simulink model "HW3"  (R2023b)
settings: Solver=VariableStepAuto  StartTime=0.0  StopTime=100  FixedStep=0.5  RelTol=1e-3
settings Model: Creator=ArshiaGosh  LastModifiedBy=ArshiaGosh

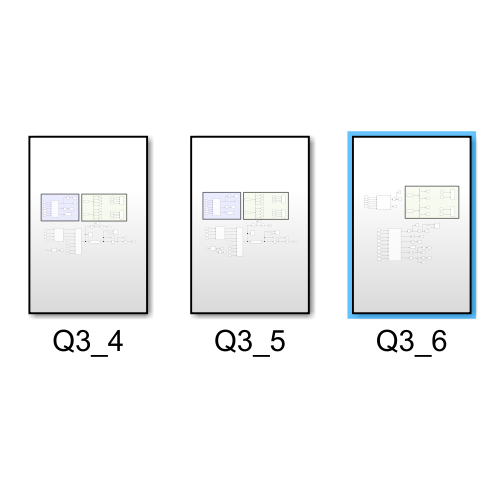
[thumbnail: Simulink's stored preview of the top-level diagram]
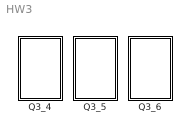
== system HW3 ==
  Q3_4 : Subsystem
  Q3_5 : Subsystem
  Q3_6 : Subsystem

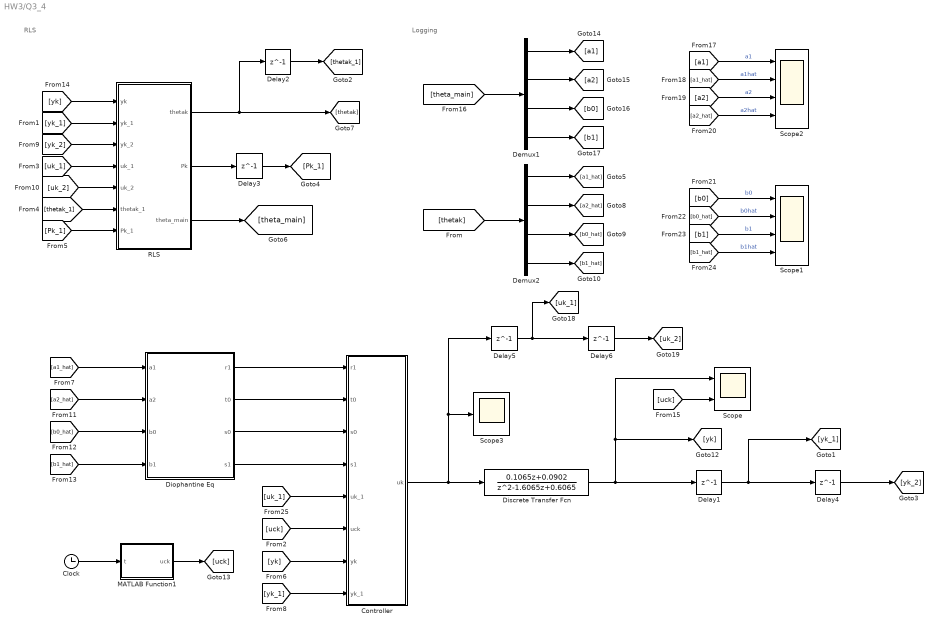
== system HW3/Q3_4 ==
  note: Logging
  note: RLS
  Clock : Clock
  Controller : MATLAB Function  TreatAsAtomicUnit=on
  Delay{1,4..6} (4 alike) : Delay  DelayLength=1
  Delay2 : Delay  DelayLength=1  InitialCondition=[0;0;0.01;0.2]
  Delay3 : Delay  DelayLength=1  InitialCondition=[100 0 0 0;0 100 0 0;0 0 1 0;0 0 0 1]
  Demux1 : Demux
  Demux2 : Demux
  Diophantine Eq : MATLAB Function  TreatAsAtomicUnit=on
  Discrete Transfer Fcn : DiscreteTransferFcn  Numerator=[0.1065 0.0902]  Denominator=[1 -1.6065 0.6065]
  MATLAB Function1 : MATLAB Function  TreatAsAtomicUnit=on
  RLS : MATLAB Function  TreatAsAtomicUnit=on
  Scope : Scope  NumInputPorts=2
  Scope1 : Scope  NumInputPorts=4
  Scope2 : Scope  NumInputPorts=4
  Scope3 : Scope
  wires:
  [yk_2] -> RLS/3(yk_2)
  Discrete Transfer Fcn/1 -> Delay1/1, [yk], Scope/1
  Delay4/1 -> [yk_2]
  [b0_hat] -> Diophantine Eq/3(b0)
  [a1_hat] -> Diophantine Eq/1(a1)
  [b1_hat] -> Diophantine Eq/4(b1)
  RLS/3(theta_main) -> [theta_main]
  [Pk_1] -> RLS/7(Pk_1)
  Delay2/1 -> [thetak_1]
  [yk_1] -> RLS/2(yk_1)
  RLS/1(thetak) -> Delay2/1, [thetak]
  Delay3/1 -> [Pk_1]
  [uck] -> Scope/2
  [uk_2] -> RLS/5(uk_2)
  Delay1/1 -> Delay4/1, [yk_1]
  Demux1/2 -> [a2]
  [thetak_1] -> RLS/6(thetak_1)
  [a2_hat] -> Diophantine Eq/2(a2)
  RLS/2(Pk) -> Delay3/1
  Demux1/3 -> [b0]
  Demux1/4 -> [b1]
  [uk_1] -> RLS/4(uk_1)
  [theta_main] -> Demux1/1
  Demux1/1 -> [a1]
  [a1] -> Scope2/1  "a1"
  [a1_hat] -> Scope2/2  "a1hat"
  [a2] -> Scope2/3  "a2"
  [a2_hat] -> Scope2/4  "a2hat"
  [b0] -> Scope1/1  "b0"
  [b0_hat] -> Scope1/2  "b0hat"
  [b1_hat] -> Scope1/4  "b1hat"
  [b1] -> Scope1/3  "b1"
  Diophantine Eq/3(s0) -> Controller/3(s0)
  Diophantine Eq/2(t0) -> Controller/2(t0)
  Diophantine Eq/1(r1) -> Controller/1(r1)
  Diophantine Eq/4(s1) -> Controller/4(s1)
  MATLAB Function1/1(uck) -> [uck]
  Clock/1 -> MATLAB Function1/1(t)
  [uck] -> Controller/6(uck)
  [yk] -> Controller/7(yk)
  [yk_1] -> Controller/8(yk_1)
  [yk] -> RLS/1(yk)
  Delay5/1 -> Delay6/1, [uk_1]
  [uk_1] -> Controller/5(uk_1)
  Delay6/1 -> [uk_2]
  Controller/1(uk) -> Discrete Transfer Fcn/1, Scope3/1, Delay5/1
  [thetak] -> Demux2/1
  Demux2/3 -> [b0_hat]
  Demux2/4 -> [b1_hat]
  Demux2/2 -> [a2_hat]
  Demux2/1 -> [a1_hat]

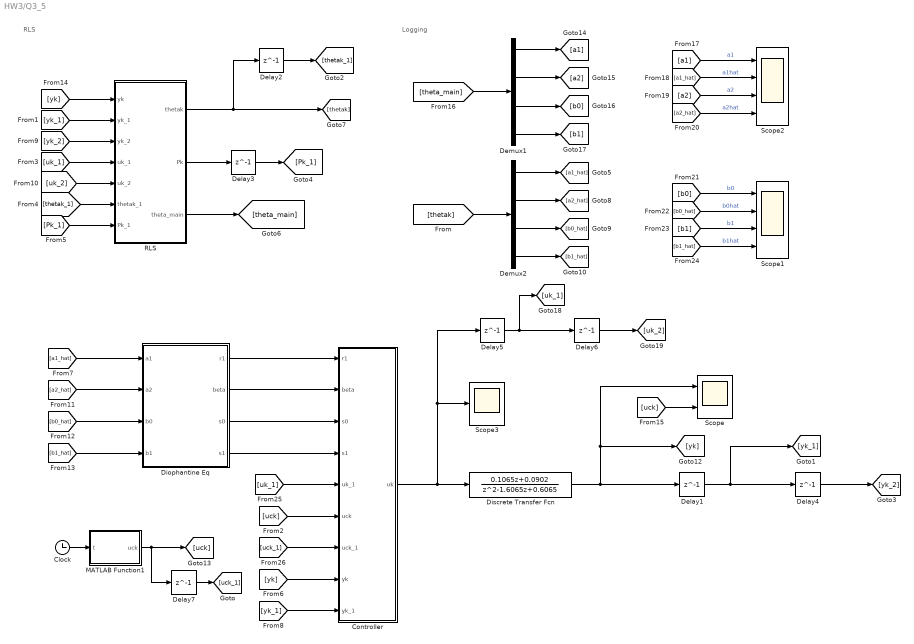
== system HW3/Q3_5 ==
  note: Logging
  note: RLS
  Clock : Clock
  Controller : MATLAB Function  TreatAsAtomicUnit=on
  Delay{1,4..7} (5 alike) : Delay  DelayLength=1
  Delay2 : Delay  DelayLength=1  InitialCondition=[0;0;0.01;0.2]
  Delay3 : Delay  DelayLength=1  InitialCondition=[100 0 0 0;0 100 0 0;0 0 1 0;0 0 0 1]
  Demux1 : Demux
  Demux2 : Demux
  Diophantine Eq : MATLAB Function  TreatAsAtomicUnit=on
  Discrete Transfer Fcn : DiscreteTransferFcn  Numerator=[0.1065 0.0902]  Denominator=[1 -1.6065 0.6065]
  MATLAB Function1 : MATLAB Function  TreatAsAtomicUnit=on
  RLS : MATLAB Function  TreatAsAtomicUnit=on
  Scope : Scope  NumInputPorts=2
  Scope1 : Scope  NumInputPorts=4
  Scope2 : Scope  NumInputPorts=4
  Scope3 : Scope
  wires:
  [yk_2] -> RLS/3(yk_2)
  Discrete Transfer Fcn/1 -> Scope/1, [yk], Delay1/1
  Delay4/1 -> [yk_2]
  [b0_hat] -> Diophantine Eq/3(b0)
  [a1_hat] -> Diophantine Eq/1(a1)
  [b1_hat] -> Diophantine Eq/4(b1)
  RLS/3(theta_main) -> [theta_main]
  [Pk_1] -> RLS/7(Pk_1)
  Delay2/1 -> [thetak_1]
  [yk_1] -> RLS/2(yk_1)
  RLS/1(thetak) -> Delay2/1, [thetak]
  Delay3/1 -> [Pk_1]
  [uck] -> Scope/2
  [uk_2] -> RLS/5(uk_2)
  Delay1/1 -> Delay4/1, [yk_1]
  Demux1/2 -> [a2]
  [thetak_1] -> RLS/6(thetak_1)
  [a2_hat] -> Diophantine Eq/2(a2)
  RLS/2(Pk) -> Delay3/1
  Demux1/3 -> [b0]
  Demux1/4 -> [b1]
  [uk_1] -> RLS/4(uk_1)
  [theta_main] -> Demux1/1
  Demux1/1 -> [a1]
  [a1] -> Scope2/1  "a1"
  [a1_hat] -> Scope2/2  "a1hat"
  [a2] -> Scope2/3  "a2"
  [a2_hat] -> Scope2/4  "a2hat"
  [b0] -> Scope1/1  "b0"
  [b0_hat] -> Scope1/2  "b0hat"
  [b1_hat] -> Scope1/4  "b1hat"
  [b1] -> Scope1/3  "b1"
  Diophantine Eq/3(s0) -> Controller/3(s0)
  Diophantine Eq/2(beta) -> Controller/2(beta)
  Diophantine Eq/1(r1) -> Controller/1(r1)
  Diophantine Eq/4(s1) -> Controller/4(s1)
  MATLAB Function1/1(uck) -> [uck], Delay7/1
  Clock/1 -> MATLAB Function1/1(t)
  [uck] -> Controller/6(uck)
  [yk] -> Controller/8(yk)
  [yk_1] -> Controller/9(yk_1)
  [yk] -> RLS/1(yk)
  Delay5/1 -> Delay6/1, [uk_1]
  [uk_1] -> Controller/5(uk_1)
  Delay6/1 -> [uk_2]
  Controller/1(uk) -> Scope3/1, Delay5/1, Discrete Transfer Fcn/1
  [thetak] -> Demux2/1
  Demux2/3 -> [b0_hat]
  Demux2/4 -> [b1_hat]
  Demux2/2 -> [a2_hat]
  Demux2/1 -> [a1_hat]
  Delay7/1 -> [uck_1]
  [uck_1] -> Controller/7(uck_1)

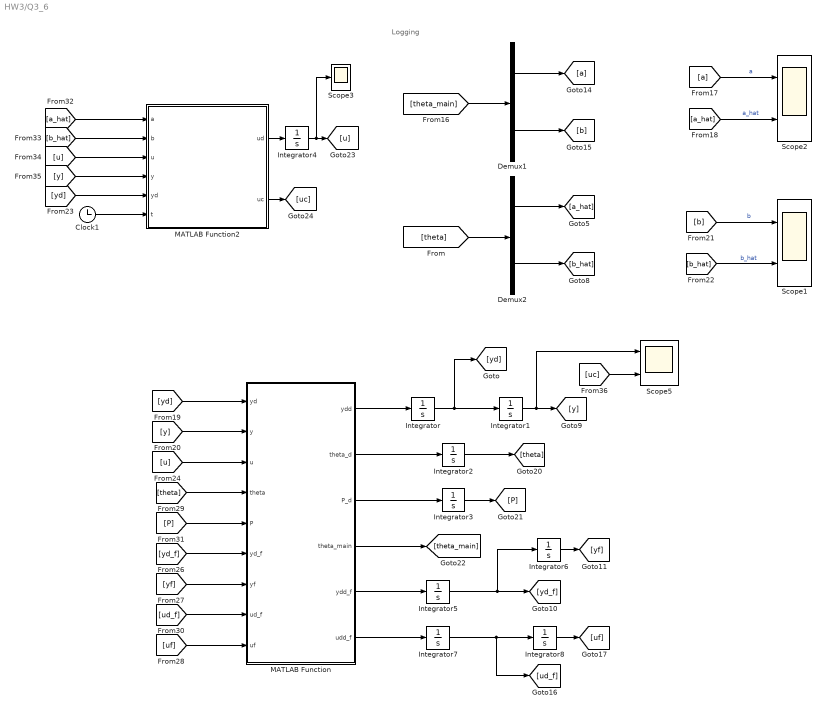
== system HW3/Q3_6 ==
  note: Logging
  Clock1 : Clock
  Demux1 : Demux  Outputs=2
  Demux2 : Demux  Outputs=2
  Integrator{,1,5..8} (6 alike) : Integrator
  Integrator2 : Integrator  InitialCondition=[2;0.2]
  Integrator3 : Integrator  InitialCondition=100*eye(2,2)
  Integrator4 : Integrator  InitialCondition=1.5
  MATLAB Function : MATLAB Function  TreatAsAtomicUnit=on
  MATLAB Function2 : MATLAB Function  TreatAsAtomicUnit=on
  Scope1 : Scope  NumInputPorts=2
  Scope2 : Scope  NumInputPorts=2
  Scope3 : Scope
  Scope5 : Scope  NumInputPorts=2
  wires:
  Demux2/1 -> [a_hat]
  Demux2/2 -> [b_hat]
  [theta] -> Demux2/1
  [b_hat] -> Scope1/2  "b_hat"
  [b] -> Scope1/1  "b"
  [a_hat] -> Scope2/2  "a_hat"
  [a] -> Scope2/1  "a"
  Demux1/1 -> [a]
  [theta_main] -> Demux1/1
  Demux1/2 -> [b]
  MATLAB Function2/2(uc) -> [uc]
  Integrator1/1 -> Scope5/1, [y]
  [a_hat] -> MATLAB Function2/1(a)
  [yd] -> MATLAB Function/1(yd)
  Integrator5/1 -> [yd_f], Integrator6/1
  Integrator/1 -> [yd], Integrator1/1
  MATLAB Function/3(P_d) -> Integrator3/1
  [b_hat] -> MATLAB Function2/2(b)
  Clock1/1 -> MATLAB Function2/6(t)
  MATLAB Function/1(ydd) -> Integrator/1
  [yd_f] -> MATLAB Function/6(yd_f)
  Integrator4/1 -> Scope3/1, [u]
  [uf] -> MATLAB Function/9(uf)
  Integrator8/1 -> [uf]
  [y] -> MATLAB Function2/4(y)
  Integrator7/1 -> Integrator8/1, [ud_f]
  [theta] -> MATLAB Function/4(theta)
  [P] -> MATLAB Function/5(P)
  Integrator6/1 -> [yf]
  [u] -> MATLAB Function/3(u)
  [y] -> MATLAB Function/2(y)
  MATLAB Function/6(udd_f) -> Integrator7/1
  [u] -> MATLAB Function2/3(u)
  MATLAB Function2/1(ud) -> Integrator4/1
  Integrator2/1 -> [theta]
  MATLAB Function/4(theta_main) -> [theta_main]
  MATLAB Function/2(theta_d) -> Integrator2/1
  [yf] -> MATLAB Function/7(yf)
  [ud_f] -> MATLAB Function/8(ud_f)
  [yd] -> MATLAB Function2/5(yd)
  Integrator3/1 -> [P]
  MATLAB Function/5(ydd_f) -> Integrator5/1
  [uc] -> Scope5/2

== matlab function HW3/Q3_5/MATLAB Function1 ==
  data: t input; uck output
function uck = fcn(t)
if t>=0 && t<25
    uck=1;
elseif t>=25 && t<50
    uck=-1;
elseif t>=50 && t<75
    uck=1;
else
    uck=-1;
end

== matlab function HW3/Q3_5/RLS ==
  data: yk input; yk_1 input; yk_2 input; uk_1 input; uk_2 input; thetak_1 input; Pk_1 input; thetak output; Pk output; theta_main output
function [thetak,Pk,theta_main] = fcn(yk, yk_1,yk_2,uk_1,uk_2,thetak_1,Pk_1)
a1 = -1.6065;
a2 = 0.6065;
b0 = 0.1065;
b1 = 0.0902;
theta_main=[a1;a2;b0;b1];

%estimate
phi = [-yk_1;-yk_2;uk_1;uk_2];
Kk = Pk_1*phi*pinv(1+phi'*Pk_1*phi);
Pk = (eye(4,4)-Kk*phi')*Pk_1;
thetak = thetak_1+Kk*(yk-phi'*thetak_1);

== matlab function HW3/Q3_6/MATLAB Function ==
  data: yd input; y input; u input; ydd output; theta input; P input; theta_d output; P_d output; theta_main output; yd_f input; yf input; ud_f input; uf input; ydd_f output; udd_f output
function [ydd,theta_d,P_d,theta_main,ydd_f,udd_f] = fcn(yd,y,u,theta,P,yd_f,yf,ud_f,uf)
%model dynamic
alpha=.2;
a=1;
b=1;
a0=2;
zeta=0.7;
w=1;
theta_main=[a;b];
ydd=-a*yd+b*u;

%filtred model
ydd_f=-2*zeta*w*yd_f-w^2*yf+y;
udd_f=-2*zeta*w*ud_f-w^2*uf+u;

%estimate of parameter
phi=[-yd_f uf]';
P_d=alpha*P-P*phi*phi'*P;
theta_d=P*phi*(ydd_f-phi'*theta);

== matlab function HW3/Q3_6/MATLAB Function2 ==
  data: a input; b input; u input; ud output; y input; yd input; t input; uc output
function [ud,uc] = fcn(a,b,u,y,yd,t)
a0=2;
zeta=0.7;
w=1;
r1=2*zeta*w+a0-a;
t0=w^2/b;
s0=(a0*2*zeta*w+w^2-a*r1)/b;
s1=(w^2*a0)/b;

%input
if t>=0 && t<25
    uc=1;
elseif t>=25 && t<50
    uc=-1;
elseif t>=50 && t<75
    uc=1;
else
    uc=-1;
end
ucd=0;

%controller
ud=-s0*yd-s1*y+ucd*t0+uc*t0*a0-r1*u

== matlab function HW3/Q3_4/Diophantine Eq ==
  data: r1 output; t0 output; s0 output; s1 output; a1 input; a2 input; b0 input; b1 input
function [r1,t0,s0,s1]   = fcn(a1,a2,b0,b1)
am1=-1.3205;
am2=0.4966;
bm0=0.1761;
r1 = b1/b0;
t0 = bm0/b0;
s0 = (am1-a1)/b0;
s1 = (am2-a2)/b0;

== matlab function HW3/Q3_4/RLS ==
  data: yk input; yk_1 input; yk_2 input; uk_1 input; uk_2 input; thetak_1 input; Pk_1 input; thetak output; Pk output; theta_main output
function [thetak,Pk,theta_main] = fcn(yk, yk_1,yk_2,uk_1,uk_2,thetak_1,Pk_1)
a1 = -1.6065;
a2 = 0.6065;
b0 = 0.1065;
b1 = 0.0902;
theta_main=[a1;a2;b0;b1];

%estimate
phi = [-yk_1;-yk_2;uk_1;uk_2];
Kk = Pk_1*phi*pinv(1+phi'*Pk_1*phi);
Pk = (eye(4,4)-Kk*phi')*Pk_1;
thetak = thetak_1+Kk*(yk-phi'*thetak_1);

== matlab function HW3/Q3_5/Controller ==
  data: r1 input; uk output; beta input; s0 input; s1 input; uk_1 input; uck input; uck_1 input; yk input; yk_1 input
function uk = fcn(r1,beta, s0,s1,uk_1, uck, uck_1,yk,yk_1)
a0=0;
uk= - uk_1*r1+beta*uck+beta*a0*uck_1-s0*yk-s1*yk_1;

== matlab function HW3/Q3_5/Diophantine Eq ==
  data: r1 output; beta output; s0 output; s1 output; a1 input; a2 input; b0 input; b1 input
function [r1,beta,s0,s1]   = fcn(a1,a2,b0,b1)
am1=-1.3205;
am2=0.4966;
bm0=0.1761;
beta=(1+am1+am2)/(b0+b1);
bm0=beta*b0;
a0=0;
r1=(a0*am2*b0^2+(a2-am2-a0*am1)*b0*b1+(a0+am1-a1)*b1^2)/(b1^2-a1*b0*b1+a2*b0^2);
s0=(b1*(a0*am1-a2-am1*a1+a1^2+am2-a1*a0)+b0*(am1*a2-a1*a2-a0*am2+a0*a2))/(b1^2-a1*b0*b1+a2*b0^2);
s1=(b1*(a1*a2-am1*a2+a0*am2-a0*a2)+b0*(a2*am2-a2^2-a0*am2*a1-a0*a2*am1))/(b1^2-a1*b0*b1+a2*b0^2);

== matlab function HW3/Q3_4/Controller ==
  data: r1 input; uk output; t0 input; s0 input; s1 input; uk_1 input; uck input; yk input; yk_1 input
function uk = fcn(r1,t0,s0,s1,uk_1, uck,yk,yk_1)

uk = -r1*uk_1 + t0*uck - s0*yk - s1*yk_1;

== matlab function HW3/Q3_4/MATLAB Function1 ==
  data: t input; uck output
function uck = fcn(t)
if t>=0 && t<25
    uck=1;
elseif t>=25 && t<50
    uck=-1;
elseif t>=50 && t<75
    uck=1;
else
    uck=-1;
end
